simulink subsystem "Car2Kep"  (R2024b)
settings: Solver=VariableStepAuto  StartTime=0.0  StopTime=10.0  RelTol=1e-3
libraries: simulink x5, matrix_library x3, vrlib x1
settings Model: Creator=marco  LastModifiedBy=ferru

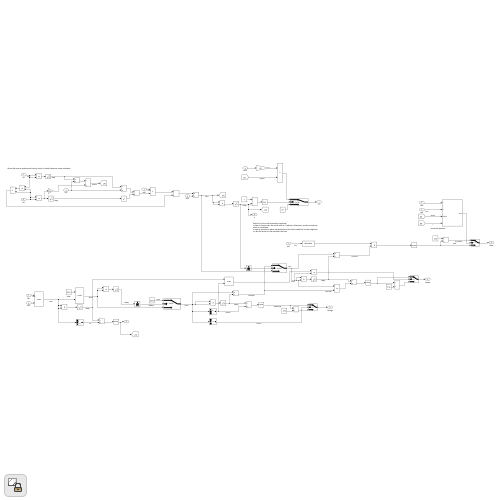
[thumbnail: Simulink's stored preview of the top-level diagram]
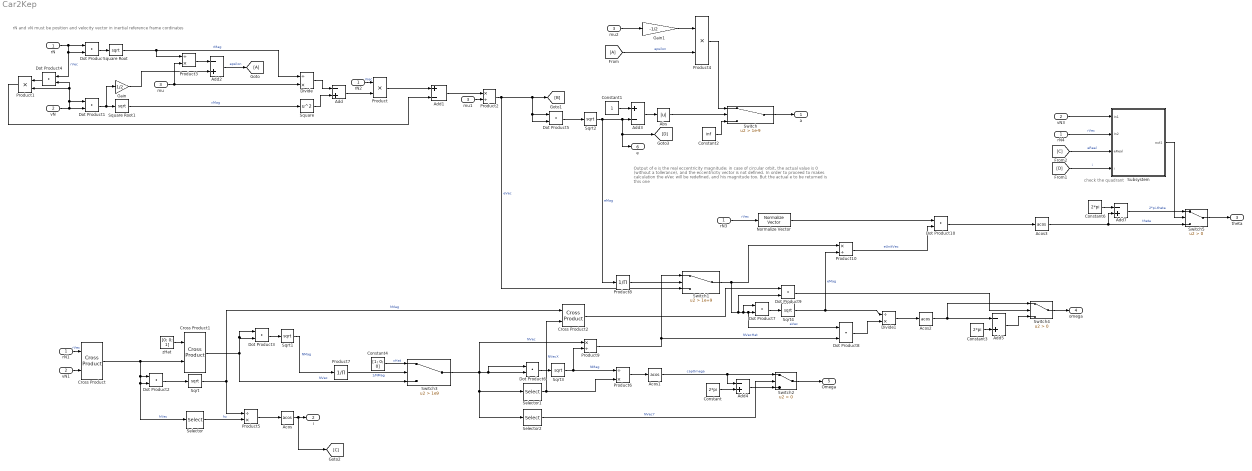
== system Car2Kep ==
  note: check the quadrant
  note: Output of e is the real eccentricity magnitude:
      | in case of circular orbit, the actual value is 0 (without a tollerance), and the eccentricity vector is not defined.
      | In order to proceed to makes calculation the eVec will be redefined, and his magnitude too. But the actual e to be returned is this one
  note: rN and vN must be position and velocity vector in inertial reference frame cordinates
  rN : Inport
  vN : Inport  Port=2
  mu : Inport  Port=3
  Abs : Abs  SaturateOnIntegerOverflow=off
  Acos{,1..3} (4 alike) : Trigonometry  Operator=acos
  Add{,2,4..5,7} (5 alike) : Sum  Inputs=-+
  Add1 : Sum  Inputs=+-
  Add3 : Sum  Inputs=+-
  Constant : Constant  Value=2*pi
  Constant1 : Constant
  Constant2 : Constant  Value=inf
  Constant3 : Constant  Value=2*pi
  Constant4 : Constant  Value=[1; 0; 0]  VectorParams1D=off
  Constant6 : Constant  Value=2*pi
  Cross Product : matrix_library/Cross Product
  Cross Product1 : matrix_library/Cross Product
  Cross Product2 : matrix_library/Cross Product
  Divide : Product  Inputs=/*
  Divide1 : Product  Inputs=/*
  Dot Product{,1..9} (10 alike) : DotProduct  OutDataTypeStr=Inherit: Inherit via internal rule
  Dot Product10 : DotProduct  OutMin=-1  OutMax=1  OutDataTypeStr=Inherit: Inherit via internal rule
  From : From
  Gain : Gain  Gain=1/2
  Gain1 : Gain  Gain=-1/2
  Goto : Goto
  Normalize Vector : vrlib/Utilities/Normalize Vector  maxzero=0
  Product : Product
  Product1 : Product
  Product10 : Product  Inputs=*/
  Product2 : Product  Inputs=*/
  Product3 : Product  Inputs=/*
  Product4 : Product
  Product5 : Product  Inputs=/*
  Product6 : Product  Inputs=/*
  Product7 : Product  Inputs=/
  Product8 : Product  Inputs=/
  Product9 : Product  Inputs=*/
  Selector : Selector  InputPortWidth=3  IndexOptions=Index vector (dialog)  Indices=3  OutputSizes=1
  Selector1 : Selector  InputPortWidth=3  IndexOptions=Index vector (dialog)  Indices=1  OutputSizes=1
  Selector2 : Selector  InputPortWidth=3  IndexOptions=Index vector (dialog)  Indices=2  OutputSizes=1
  Sqrt{,1..4} (5 alike) : Sqrt
  Square : Math  Operator=square
  Square Root : Sqrt
  Square Root1 : Sqrt
  Subsystem : Subsystem
  Switch : Switch  Criteria=u2 > Threshold  Threshold=1e-9  SaturateOnIntegerOverflow=off  InputSameDT=off
  Switch1 : Switch  Criteria=u2 > Threshold  Threshold=1e+9  SaturateOnIntegerOverflow=off  InputSameDT=off
  Switch2 : Switch  Criteria=u2 > Threshold  SaturateOnIntegerOverflow=off  InputSameDT=off
  Switch3 : Switch  Criteria=u2 > Threshold  Threshold=1e9  SaturateOnIntegerOverflow=off  InputSameDT=off
  Switch4 : Switch  Criteria=u2 > Threshold  SaturateOnIntegerOverflow=off  InputSameDT=off
  Switch5 : Switch  Criteria=u2 > Threshold  SaturateOnIntegerOverflow=off  InputSameDT=off
  mu1 : InportShadow  Port=3
  mu2 : InportShadow  Port=3
  rN{1..4} (4 alike) : InportShadow
  vN1 : InportShadow  Port=2
  vN3 : InportShadow  Port=2
  zHat : Constant  Value=[0; 0; 1]  VectorParams1D=off
  a : Outport
  i : Outport  Port=2
  theta : Outport  Port=3
  omega : Outport  Port=4
  Omega : Outport  Port=5
  e : Outport  Port=6
  wires:
  rN/1 -> Dot Product/1, Dot Product4/1, Dot Product/2  "rVec"
  Dot Product/1 -> Square Root/1
  Square Root/1 -> Product3/1, Divide/1  "rMag"
  Dot Product1/1 -> Square Root1/1, Gain/1
  vN/1 -> Dot Product1/2, Dot Product4/2, Product1/2, Dot Product1/1
  Square Root1/1 -> Square/1  "vMag"
  Cross Product/1 -> Dot Product2/1, Dot Product2/2, Selector/1, Cross Product1/2  "hVec"
  Dot Product2/1 -> Sqrt/1
  zHat/1 -> Cross Product1/1
  Cross Product1/1 -> Switch3/3, Dot Product3/2, Dot Product3/1  "NVec"
  Dot Product3/1 -> Sqrt1/1
  Sqrt/1 -> Product5/1, Cross Product2/1  "hMag"
  Sqrt1/1 -> Product7/1  "NMag"
  mu/1 -> Product3/2, Divide/2
  rN1/1 -> Cross Product/1  "rVec"
  vN1/1 -> Cross Product/2
  Square/1 -> Add/2
  Divide/1 -> Add/1
  Add/1 -> Product/2
  Product/1 -> Add1/1
  Dot Product4/1 -> Product1/1
  Product1/1 -> Add1/2
  Add1/1 -> Product2/1
  mu1/1 -> Product2/2
  Product2/1 -> [B], Dot Product5/1, Dot Product5/2, Switch1/3  "eVec"
  rN2/1 -> Product/1  "rVec"
  Dot Product5/1 -> Sqrt2/1
  Sqrt2/1 -> Add3/2, [D], e/1, Product8/1  "eMag"
  Gain/1 -> Add2/2
  Product3/1 -> Add2/1
  Add2/1 -> Goto/1  "epsilon"
  Constant1/1 -> Add3/1
  Add3/1 -> Abs/1
  Product4/1 -> Switch/1
  mu2/1 -> Gain1/1
  Gain1/1 -> Product4/1
  From/1 -> Product4/2  "epsilon"
  Constant2/1 -> Switch/3
  Selector/1 -> Product5/2  "hz"
  Product5/1 -> Acos/1
  Acos/1 -> i/1, [C]
  Abs/1 -> Switch/2
  Switch/1 -> a/1
  Acos1/1 -> Add4/1, Switch2/1  "capOmega"
  Selector1/1 -> Product6/2, Cross Product2/2  "NVecX"
  Product6/1 -> Acos1/1
  Selector2/1 -> Switch2/2  "NVecY"
  Switch2/1 -> Omega/1
  Constant/1 -> Add4/2
  Add4/1 -> Switch2/3
  Product7/1 -> Switch3/2  "1/NMag"
  Constant4/1 -> Switch3/1  "xHat"
  Switch3/1 -> Dot Product6/1, Dot Product6/2, Selector1/1, Selector2/1, Product9/1  "NVec"
  Sqrt3/1 -> Product6/1, Product9/2  "NMag"
  Dot Product6/1 -> Sqrt3/1
  Product8/1 -> Switch1/2
  Product9/1 -> Dot Product8/2, Switch1/1  "NVecHat"
  Switch1/1 -> Dot Product7/2, Dot Product8/1, Dot Product7/1, Dot Product9/2, Product10/1  "eVec"
  Dot Product7/1 -> Sqrt4/1
  Sqrt4/1 -> Divide1/1, Product10/2  "eMag"
  Dot Product8/1 -> Divide1/2
  Divide1/1 -> Acos2/1
  Acos2/1 -> Switch4/1, Add5/1
  Switch4/1 -> omega/1
  Constant3/1 -> Add5/2
  Add5/1 -> Switch4/3
  Product10/1 -> Dot Product10/2  "eUnitVec"
  Dot Product10/1 -> Acos3/1
  Acos3/1 -> Switch5/3, Add7/2  "theta"
  Add7/1 -> Switch5/1  "2*pi-theta"
  Constant6/1 -> Add7/1
  vN3/1 -> Subsystem/1(In1)
  rN4/1 -> Subsystem/2(In2)  "rVec"
  [C] -> Subsystem/3(eReal)  "eReal"
  [D] -> Subsystem/4(i)  "i"
  Subsystem/1(out1) -> Switch5/2
  Switch5/1 -> theta/1
  rN3/1 -> Normalize Vector/1  "rVec"
  Normalize Vector/1 -> Dot Product10/1
  Cross Product2/1 -> Dot Product9/1
  Dot Product9/1 -> Switch4/2

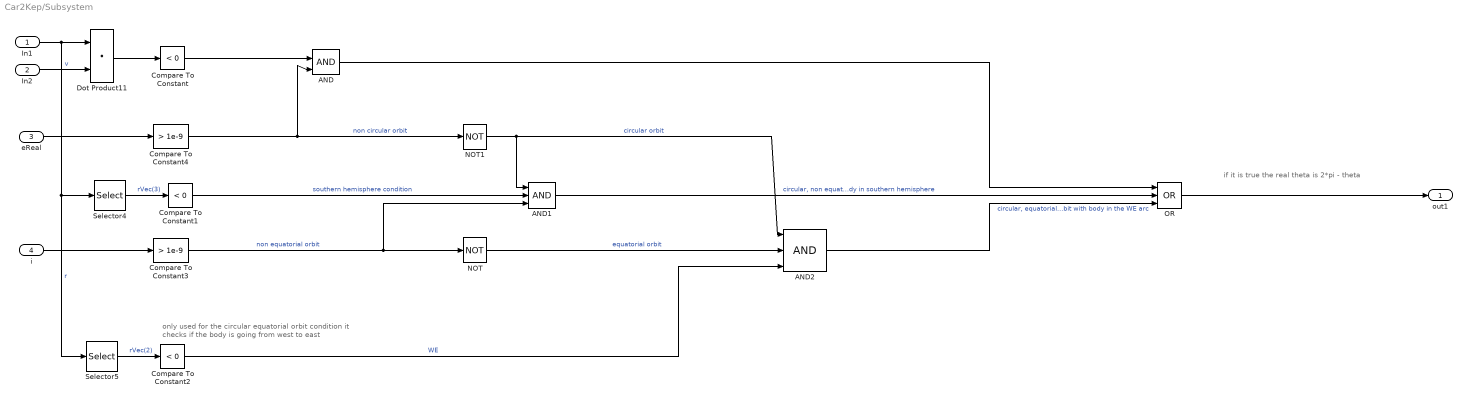
== system Car2Kep/Subsystem ==
  note: only used for the circular equatorial orbit condition
      | it checks if the body is going from west to east
  note: if it is true the real theta is 2*pi - theta
  In1 : Inport
  In2 : Inport  Port=2
  eReal : Inport  Port=3
  i : Inport  Port=4
  AND : Logic  IconShape=distinctive  AllPortsSameDT=off  OutDataTypeStr=boolean
  AND1 : Logic  Inputs=3  IconShape=distinctive  AllPortsSameDT=off  OutDataTypeStr=boolean
  AND2 : Logic  Inputs=3  IconShape=distinctive  AllPortsSameDT=off  OutDataTypeStr=boolean
  Compare To Constant : simulink/Logic and Bit Operations/Compare To Constant  relop=<  const=0  OutDataTypeStr=boolean
  Compare To Constant1 : simulink/Logic and Bit Operations/Compare To Constant  relop=<  const=0  OutDataTypeStr=boolean
  Compare To Constant2 : simulink/Logic and Bit Operations/Compare To Constant  relop=<  const=0  OutDataTypeStr=boolean
  Compare To Constant3 : simulink/Logic and Bit Operations/Compare To Constant  relop=>  const=1e-9  OutDataTypeStr=boolean
  Compare To Constant4 : simulink/Logic and Bit Operations/Compare To Constant  relop=>  const=1e-9  OutDataTypeStr=boolean
  Dot Product11 : DotProduct  OutDataTypeStr=Inherit: Inherit via internal rule
  NOT : Logic  Operator=NOT  IconShape=distinctive  AllPortsSameDT=off  OutDataTypeStr=boolean
  NOT1 : Logic  Operator=NOT  IconShape=distinctive  AllPortsSameDT=off  OutDataTypeStr=boolean
  OR : Logic  Operator=OR  Inputs=3  IconShape=distinctive  AllPortsSameDT=off  OutDataTypeStr=boolean
  Selector4 : Selector  InputPortWidth=3  IndexOptions=Index vector (dialog)  Indices=3  OutputSizes=1
  Selector5 : Selector  InputPortWidth=3  IndexOptions=Index vector (dialog)  Indices=2  OutputSizes=1
  out1 : Outport
  wires:
  In2/1 -> Dot Product11/2  "v"
  NOT/1 -> AND2/2  "equatorial orbit"
  eReal/1 -> Compare To Constant4/1
  i/1 -> Compare To Constant3/1
  Compare To Constant/1 -> AND/1
  Selector5/1 -> Compare To Constant2/1  "rVec(2)"
  AND/1 -> OR/1
  OR/1 -> out1/1
  AND1/1 -> OR/2  "circular, non equatorial orbit with body in southern hemisphere"
  Compare To Constant1/1 -> AND1/2  "southern hemisphere condition"
  Compare To Constant3/1 -> NOT/1, AND1/3  "non equatorial orbit"
  Compare To Constant2/1 -> AND2/3  "WE"
  Compare To Constant4/1 -> NOT1/1, AND/2  "non circular orbit"
  AND2/1 -> OR/3  "circular, equatorial orbit with body in the WE arc"
  In1/1 -> Selector5/1, Selector4/1, Dot Product11/1  "r"
  Selector4/1 -> Compare To Constant1/1  "rVec(3)"
  NOT1/1 -> AND2/1, AND1/1  "circular orbit"
  Dot Product11/1 -> Compare To Constant/1
